simulink model "SPMS_Dashboard_Sim"  (R2025b)
settings: Solver=ode45  StartTime=0.0  StopTime=20  RelTol=1e-3
settings Model: Creator=acer  LastModifiedBy=acer

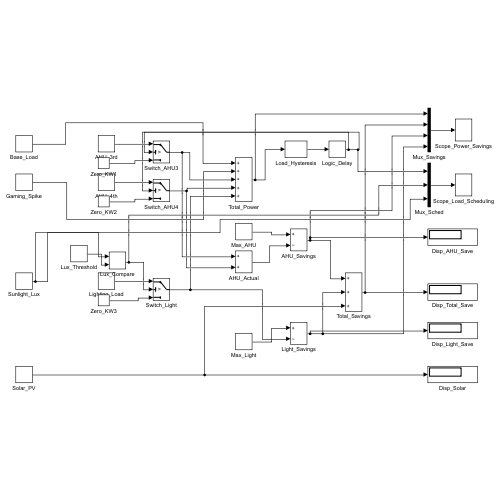
[thumbnail: Simulink's stored preview of the top-level diagram]
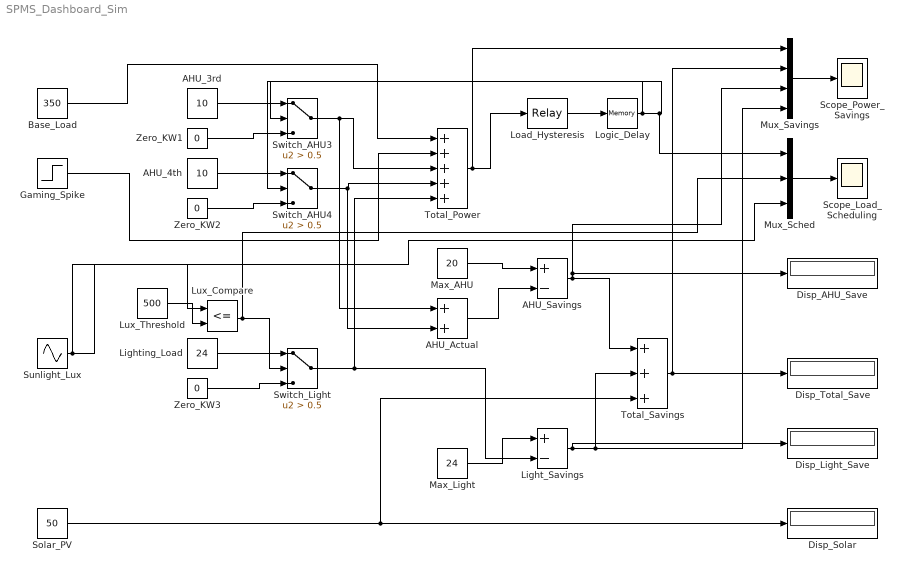
== system SPMS_Dashboard_Sim ==
  AHU_3rd : Constant  Value=10
  AHU_4th : Constant  Value=10
  AHU_Actual : Sum
  AHU_Savings : Sum  Inputs=+-
  Base_Load : Constant  Value=350
  Disp_AHU_Save : Display
  Disp_Light_Save : Display
  Disp_Solar : Display
  Disp_Total_Save : Display
  Gaming_Spike : Step  Time=5  After=220  SampleTime=0
  Light_Savings : Sum  Inputs=+-
  Lighting_Load : Constant  Value=24
  Load_Hysteresis : Relay  OnSwitchValue=600  OffSwitchValue=580  OnOutputValue=0  OffOutputValue=1
  Logic_Delay : Memory
  Lux_Compare : RelationalOperator  Operator=<=  OutDataTypeStr=boolean  RndMeth=Simplest  InputSameDT=off
  Lux_Threshold : Constant  Value=500
  Max_AHU : Constant  Value=20
  Max_Light : Constant  Value=24
  Mux_Savings : Mux
  Mux_Sched : Mux  Inputs=3
  Scope_Load_Scheduling : Scope
  Scope_Power_Savings : Scope
  Solar_PV : Constant  Value=50
  Sunlight_Lux : Sin  Amplitude=1000  Frequency=0.2  SampleTime=0
  Switch_AHU3 : Switch  Criteria=u2 > Threshold  Threshold=0.5  SaturateOnIntegerOverflow=off  InputSameDT=off
  Switch_AHU4 : Switch  Criteria=u2 > Threshold  Threshold=0.5  SaturateOnIntegerOverflow=off  InputSameDT=off
  Switch_Light : Switch  Criteria=u2 > Threshold  Threshold=0.5  SaturateOnIntegerOverflow=off  InputSameDT=off
  Total_Power : Sum  Inputs=+++++
  Total_Savings : Sum  Inputs=+++
  Zero_KW1 : Constant  Value=0
  Zero_KW2 : Constant  Value=0
  Zero_KW3 : Constant  Value=0
  wires:
  AHU_3rd/1 -> Switch_AHU3/1
  Zero_KW1/1 -> Switch_AHU3/3
  AHU_4th/1 -> Switch_AHU4/1
  Zero_KW2/1 -> Switch_AHU4/3
  Lighting_Load/1 -> Switch_Light/1
  Zero_KW3/1 -> Switch_Light/3
  Base_Load/1 -> Total_Power/1
  Gaming_Spike/1 -> Total_Power/2
  Switch_AHU3/1 -> Total_Power/3, AHU_Actual/1
  Switch_AHU4/1 -> Total_Power/4, AHU_Actual/2
  Switch_Light/1 -> Total_Power/5, Light_Savings/2
  Total_Power/1 -> Load_Hysteresis/1, Mux_Savings/1
  Load_Hysteresis/1 -> Logic_Delay/1
  Logic_Delay/1 -> Switch_AHU3/2, Mux_Sched/1, Switch_AHU4/2
  Sunlight_Lux/1 -> Lux_Compare/1, Mux_Sched/3
  Lux_Threshold/1 -> Lux_Compare/2
  Lux_Compare/1 -> Switch_Light/2, Mux_Sched/2
  Max_AHU/1 -> AHU_Savings/1
  AHU_Actual/1 -> AHU_Savings/2
  Max_Light/1 -> Light_Savings/1
  AHU_Savings/1 -> Disp_AHU_Save/1, Mux_Savings/3, Total_Savings/1
  Light_Savings/1 -> Total_Savings/2, Mux_Savings/4, Disp_Light_Save/1
  Solar_PV/1 -> Total_Savings/3, Disp_Solar/1
  Total_Savings/1 -> Disp_Total_Save/1, Mux_Savings/2
  Mux_Savings/1 -> Scope_Power_Savings/1
  Mux_Sched/1 -> Scope_Load_Scheduling/1
